simulink model "lab2"  (R2025b)
settings: Solver=FixedStepAuto  StartTime=0.0  StopTime=10.0  FixedStep=0.001  RelTol=1e-3
undefined symbols (not defined in the file): A, a01, a02, B, C, D, K, k1, k2, ksi, T1
settings Model: Creator=Nickolay  LastModifiedBy=Nickolay

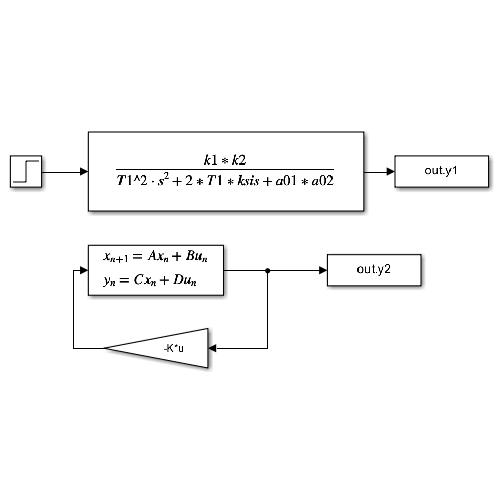
[thumbnail: Simulink's stored preview of the top-level diagram]
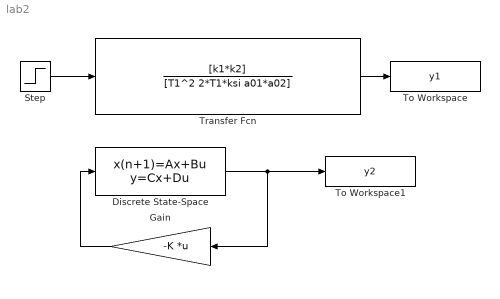
== system lab2 ==
  Discrete State-Space : DiscreteStateSpace  A=A  B=B  C=C  D=D  InitialCondition=[1;0]
  Gain : Gain  Gain=-K  Multiplication=Matrix(K*u)
  Step : Step  SampleTime=0
  To Workspace : ToWorkspace  VariableName=y1  SaveFormat=Timeseries  SampleTime=-1
  To Workspace1 : ToWorkspace  VariableName=y2  SaveFormat=Timeseries  SampleTime=-1
  Transfer Fcn : TransferFcn  Numerator=[k1*k2]  Denominator=[T1^2 2*T1*ksi a01*a02]
  wires:
  Step/1 -> Transfer Fcn/1
  Transfer Fcn/1 -> To Workspace/1
  Discrete State-Space/1 -> Gain/1, To Workspace1/1
  Gain/1 -> Discrete State-Space/1
